simulink model "mavsim_manager_video"  (R2025a)
settings: Solver=ode45  StartTime=0.0  StopTime=inf  RelTol=1e-3  EnableMultiTasking=on
InitFcn:
  | param_chap11
undefined symbols (not defined in the file): autopilot, drawEnvironment, estimate_states, fym, gps, P, path_manager, path_planner_chap11, seguimiento, sensors, true_states
libraries: simulink x4
settings Model: Creator=beard  LastModifiedBy=anton
settings SolverCC: AlgebraicLoopSolver=TrustRegion
settings DataIOCC: LimitDataPoints=on  SaveFormat=Array  SignalLoggingSaveFormat=ModelDataLogs  ReturnWorkspaceOutputs=off
settings OptimizationCC: ExpressionDepthLimit=2147483647.0  InitFltsAndDblsToZero=on  LifeSpan=inf
settings DebuggingCC: UnderspecifiedInitializationDetection=Classic  MergeDetectMultiDrivingBlocksExec=none  SolverPrmCheckMsg=warning  FcnCallInpInsideContextMsg=warning  UnconnectedInputMsg=warning  UnconnectedOutputMsg=warning  UnconnectedLineMsg=warning  StateNameClashWarn=warning  SFUnexpectedBacktrackingDiag=warning  SFNoUnconditionalDefaultTransitionDiag=warning  ArithmeticOperatorsInVariantConditions=warning
settings HardwareCC: ProdBitPerPointer=32.0  ProdBitPerSizeT=32.0  ProdBitPerPtrDiffT=32.0  ProdLargestAtomicFloat=None  ProdIntDivRoundTo=Undefined  ProdEndianess=Unspecified  ProdWordSize=32.0  ProdHWDeviceType=32-bit Generic
settings ModelReferenceCC: EnableRefExpFcnMdlSchedulingChecks=on  PropagateSignalLabelsOutOfModel=off
settings SFSimCC: SimUseLocalCustomCode=off  SimParseCustomCode=off  CustomCodeUndefinedFunction=UseInterfaceOnly
settings RTWCC: RTWUseLocalCustomCode=off  GPUComputeCapability=3.5  DLArmComputeVersion=19.05
settings CodeAppCC: StateflowObjectComments=on
settings GRTTargetCC: TargetLangStandard=C89/C90 (ANSI)  CombineOutputUpdateFcns=off  GRTInterface=on
settings ConfigComp: CovMetricSettings=dw  CovSaveCumulativeToWorkspaceVar=on  CovSaveSingleToWorkspaceVar=on  CovExternalEMLEnable=off  CovSFcnEnable=off

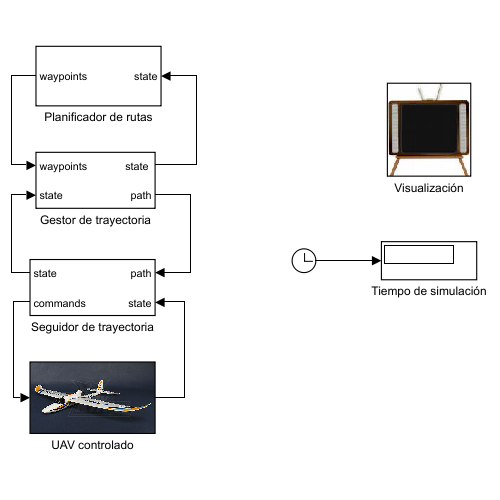
[thumbnail: Simulink's stored preview of the top-level diagram]
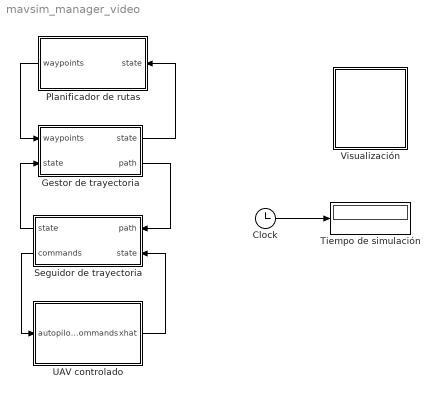
== system mavsim_manager_video ==
  Clock : Clock
  Gestor de trayectoria : Subsystem
  Planificador de rutas : Subsystem
  Seguidor de trayectoria : Subsystem
  Tiempo de simulación : Display
  UAV controlado : Subsystem
      mask Display: image(imread('uav.jpg'))
  Visualización : Subsystem
      mask Display: image(imread('tv.jpg'))
  wires:
  Clock/1 -> Tiempo de simulación/1
  Gestor de trayectoria/2(path) -> Seguidor de trayectoria/1(path)
  Seguidor de trayectoria/2(commands) -> UAV controlado/1(autopilot commands)
  UAV controlado/1(xhat) -> Seguidor de trayectoria/2(state)
  Seguidor de trayectoria/1("state ") -> Gestor de trayectoria/2(state)
  Planificador de rutas/1(waypoints) -> Gestor de trayectoria/1(waypoints)
  Gestor de trayectoria/1("state ") -> Planificador de rutas/1(state)

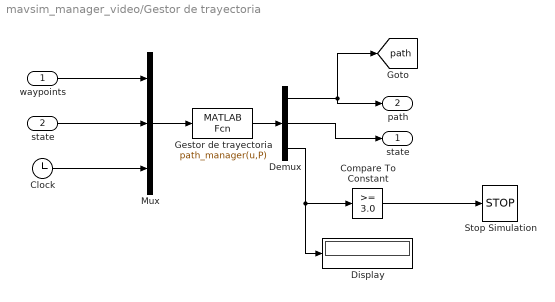
== system mavsim_manager_video/Gestor de trayectoria ==
  waypoints : Inport
  state : Inport  Port=2
  Clock : Clock
  Compare To Constant : simulink/Logic and Bit Operations/Compare To Constant  relop=>=  const=3.0  OutDataTypeStr=boolean
  Demux : Demux  Outputs=[13;17;1]
  Display : Display
  Gestor de trayectoria : MATLABFcn  MATLABFcn=path_manager(u,P)  OutputDimensions=31  SampleTime=P.Ts
  Mux : Mux  Inputs=3
  Stop Simulation : Stop
  "state " : Outport
  path : Outport  Port=2
  tag scope: path=global
  wires:
  Demux/2 -> "state "/1
  Demux/1 -> path/1, [path]
  Gestor de trayectoria/1 -> Demux/1
  waypoints/1 -> Mux/1
  state/1 -> Mux/2
  Clock/1 -> Mux/3
  Mux/1 -> Gestor de trayectoria/1
  Demux/3 -> Compare To Constant/1, Display/1
  Compare To Constant/1 -> Stop Simulation/1

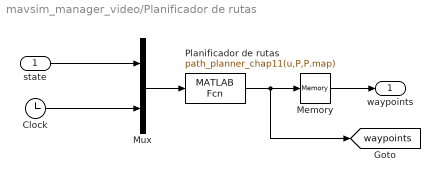
== system mavsim_manager_video/Planificador de rutas ==
  state : Inport
  Clock : Clock
  Memory : Memory
  Mux : Mux  Inputs=2
  Planificador de rutas : MATLABFcn  MATLABFcn=path_planner_chap11(u,P,P.map)  OutputDimensions=1+5*P.size_waypoint_array  SampleTime=100*P.Ts
  waypoints : Outport
  tag scope: waypoints=global
  wires:
  Mux/1 -> Planificador de rutas/1
  Clock/1 -> Mux/2
  state/1 -> Mux/1
  Planificador de rutas/1 -> Memory/1, [waypoints]
  Memory/1 -> waypoints/1

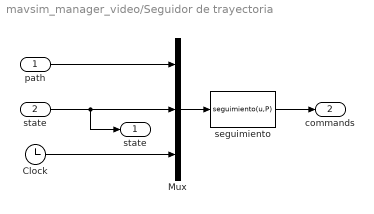
== system mavsim_manager_video/Seguidor de trayectoria ==
  path : Inport
  state : Inport  Port=2
  Clock : Clock
  Mux : Mux  Inputs=3
  seguimiento : MATLABFcn  MATLABFcn=seguimiento(u,P)  OutputDimensions=3  SampleTime=P.Ts
  "state " : Outport
  commands : Outport  Port=2
  wires:
  seguimiento/1 -> commands/1
  Mux/1 -> seguimiento/1
  path/1 -> Mux/1
  Clock/1 -> Mux/3
  state/1 -> Mux/2, "state "/1

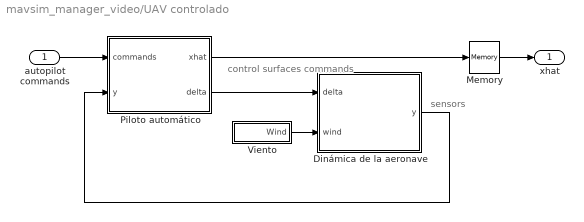
== system mavsim_manager_video/UAV controlado ==
  note: control surfaces
      | commands
  note: sensors
  autopilot commands : Inport
  Dinámica de la aeronave : Subsystem
      mask Display: image(imread('uav.jpg'))
  Memory : Memory
  Piloto automático : Subsystem
      mask Display: image(imread('pixfalcon.jpeg'))
  Viento : Subsystem
  xhat : Outport
  wires:
  Memory/1 -> xhat/1
  Piloto automático/1(xhat) -> Memory/1
  autopilot commands/1 -> Piloto automático/1(commands)
  Dinámica de la aeronave/1(y) -> Piloto automático/2(y)
  Piloto automático/2(delta) -> Dinámica de la aeronave/1(delta)
  Viento/1(Wind) -> Dinámica de la aeronave/2(wind)

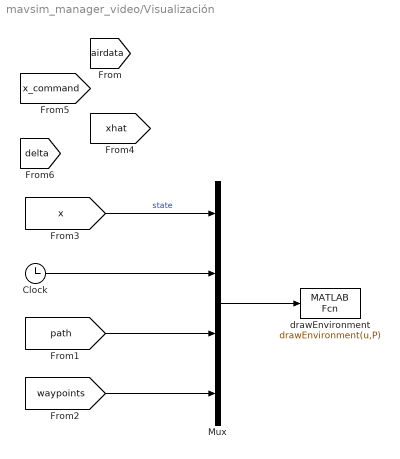
== system mavsim_manager_video/Visualización ==
  Clock : Clock
  Mux : Mux
  drawEnvironment : MATLABFcn  MATLABFcn=drawEnvironment(u,P)  OutputDimensions=0  SampleTime=0.1
  wires:
  Clock/1 -> Mux/2
  [x] -> Mux/1  "state"
  Mux/1 -> drawEnvironment/1
  [path] -> Mux/3
  [waypoints] -> Mux/4

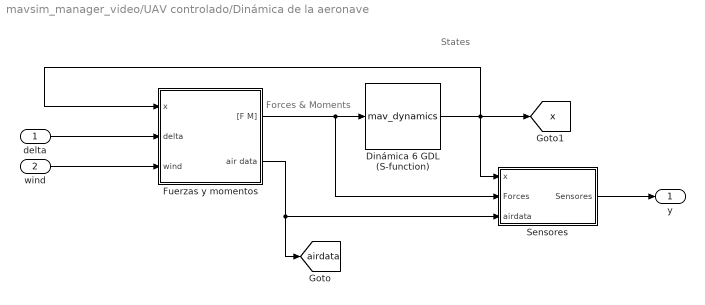
== system mavsim_manager_video/UAV controlado/Dinámica de la aeronave ==
  note: States
  note: Forces & Moments
  delta : Inport
  wind : Inport  Port=2
  Dinámica 6 GDL (S-function) : M-S-Function  FunctionName=mav_dynamics  Parameters=mass,Jx,Jy,Jz,Jxz,pn0,pe0,pd0,u0,v0,w0,phi0,theta0,psi0,p0,q0,r0  mask{mass=P.mass, Jx=P.Jx, Jy=P.Jy, Jz=P.Jz, Jxz=P.Jxz, pn0=P.pn0, pe0=P.pe0, pd0=P.pd0, u0=P.u0, v0=P.v0, w0=P.w0, phi0=P.phi0, theta0=P.theta0, psi0=P.psi0, p0=P.p0, q0=P.q0, r0=P.r0}
  Fuerzas y momentos : Subsystem
  Sensores : Subsystem
  y : Outport
  tag scope: airdata=global, x=global
  wires:
  wind/1 -> Fuerzas y momentos/3(wind)
  delta/1 -> Fuerzas y momentos/2(delta)
  Fuerzas y momentos/2(air data) -> Sensores/3(airdata), [airdata]
  Fuerzas y momentos/1("[F M]") -> Dinámica 6 GDL (S-function)/1, Sensores/2(Forces)
  Dinámica 6 GDL (S-function)/1 -> [x], Sensores/1(x), Fuerzas y momentos/1(x)
  Sensores/1(Sensores) -> y/1

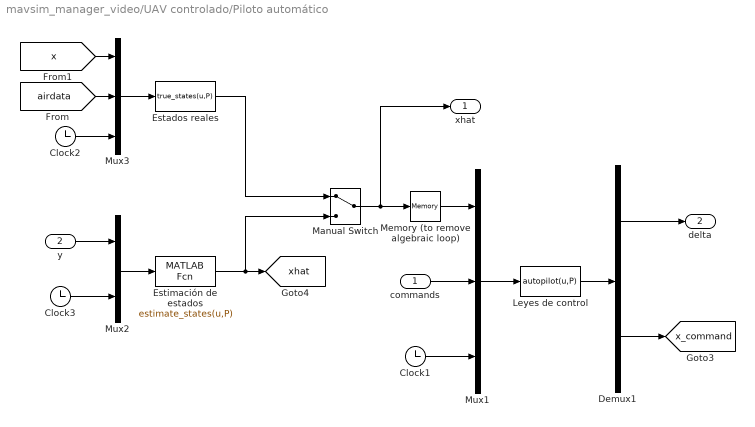
== system mavsim_manager_video/UAV controlado/Piloto automático ==
  commands : Inport
  y : Inport  Port=2
  Clock1 : Clock
  Clock2 : Clock
  Clock3 : Clock
  Demux1 : Demux  Outputs=[4;12]
  Estados reales : MATLABFcn  MATLABFcn=true_states(u,P)  OutputDimensions=19  SampleTime=P.Ts
  Estimación de estados : MATLABFcn  MATLABFcn=estimate_states(u,P)  OutputDimensions=19  SampleTime=P.Ts
  Leyes de control : MATLABFcn  MATLABFcn=autopilot(u,P)  OutputDimensions=4+12  SampleTime=P.Ts
  Manual Switch : ManualSwitch
  Memory (to remove algebraic loop) : Memory
  Mux1 : Mux  Inputs=3
  Mux2 : Mux  Inputs=2
  Mux3 : Mux  Inputs=3
  xhat : Outport
  delta : Outport  Port=2
  tag scope: x_command=global, xhat=global
  wires:
  Estimación de estados/1 -> [xhat], Manual Switch/2
  Clock3/1 -> Mux2/2
  Clock2/1 -> Mux3/3
  Clock1/1 -> Mux1/3
  [x] -> Mux3/1
  [airdata] -> Mux3/2
  Mux3/1 -> Estados reales/1
  Estados reales/1 -> Manual Switch/1
  Manual Switch/1 -> xhat/1, Memory (to remove algebraic loop)/1
  Memory (to remove algebraic loop)/1 -> Mux1/1
  y/1 -> Mux2/1
  Mux2/1 -> Estimación de estados/1
  commands/1 -> Mux1/2
  Demux1/2 -> [x_command]
  Demux1/1 -> delta/1
  Leyes de control/1 -> Demux1/1
  Mux1/1 -> Leyes de control/1

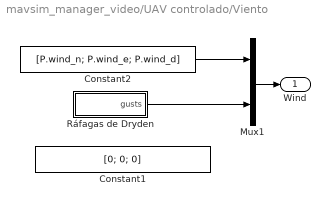
== system mavsim_manager_video/UAV controlado/Viento ==
  Constant1 : Constant  Value=[0; 0; 0]
  Constant2 : Constant  Value=[P.wind_n; P.wind_e; P.wind_d]
  Mux1 : Mux  Inputs=2
  Ráfagas de Dryden : Subsystem
  Wind : Outport
  wires:
  Mux1/1 -> Wind/1
  Constant2/1 -> Mux1/1
  Ráfagas de Dryden/1(gusts) -> Mux1/2

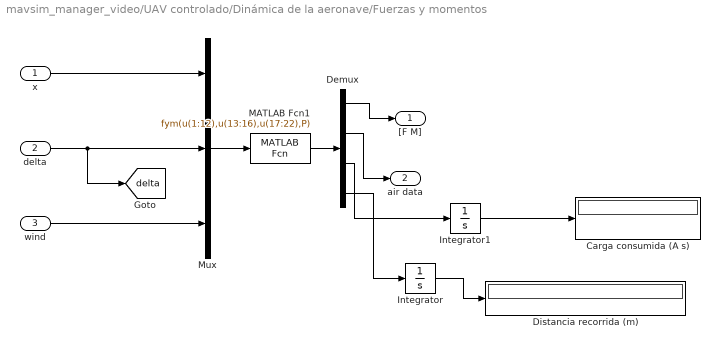
== system mavsim_manager_video/UAV controlado/Dinámica de la aeronave/Fuerzas y momentos ==
  x : Inport
  delta : Inport  Port=2
  wind : Inport  Port=3
  Carga consumida (A s) : Display
  Demux : Demux  Outputs=[6;6;1;1]
  Distancia recorrida (m) : Display
      settings: Decimation=4
  Integrator : Integrator
  Integrator1 : Integrator
  MATLAB Fcn1 : MATLABFcn  MATLABFcn=fym(u(1:12),u(13:16),u(17:22),P)  OutputDimensions=14
  Mux : Mux  Inputs=3
  "[F M]" : Outport
  air data : Outport  Port=2
  tag scope: delta=global
  wires:
  Demux/2 -> air data/1
  Mux/1 -> MATLAB Fcn1/1
  Demux/1 -> "[F M]"/1
  MATLAB Fcn1/1 -> Demux/1
  wind/1 -> Mux/3
  delta/1 -> Mux/2, [delta]
  x/1 -> Mux/1
  Demux/3 -> Integrator1/1
  Demux/4 -> Integrator/1
  Integrator/1 -> Distancia recorrida (m)/1
  Integrator1/1 -> Carga consumida (A s)/1

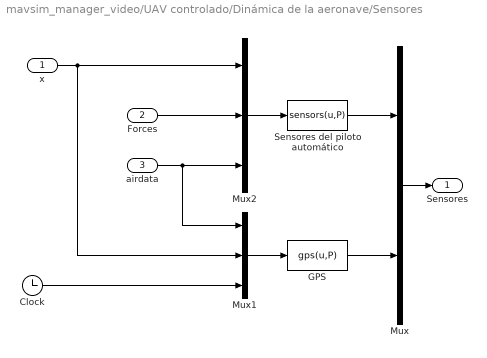
== system mavsim_manager_video/UAV controlado/Dinámica de la aeronave/Sensores ==
  x : Inport
  Forces : Inport  Port=2
  airdata : Inport  Port=3
  Clock : Clock
  GPS : MATLABFcn  MATLABFcn=gps(u,P)  OutputDimensions=5  SampleTime=P.Ts_gps
  Mux : Mux  Inputs=2
  Mux1 : Mux  Inputs=3
  Mux2 : Mux  Inputs=3
  Sensores del piloto automático : MATLABFcn  MATLABFcn=sensors(u,P)  OutputDimensions=8  SampleTime=P.Ts
  Sensores : Outport
  wires:
  x/1 -> Mux1/2, Mux2/1
  Mux/1 -> Sensores/1
  airdata/1 -> Mux1/1, Mux2/3
  Forces/1 -> Mux2/2
  Mux2/1 -> Sensores del piloto automático/1
  Clock/1 -> Mux1/3
  Mux1/1 -> GPS/1
  GPS/1 -> Mux/2
  Sensores del piloto automático/1 -> Mux/1

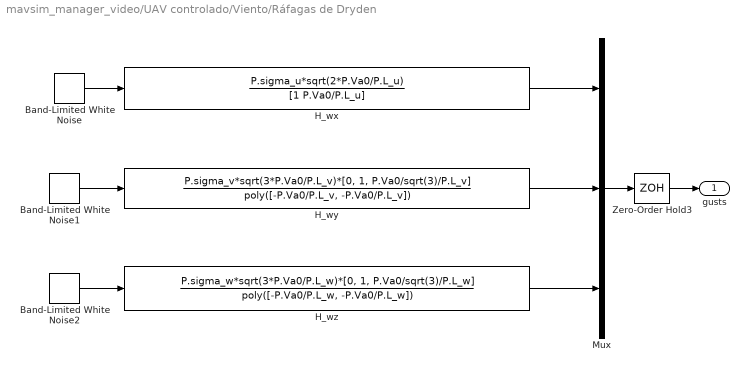
== system mavsim_manager_video/UAV controlado/Viento/Ráfagas de Dryden ==
  Band-Limited White Noise : simulink/Sources/Band-Limited White Noise  Cov=[1]  Ts=P.Ts  seed=[23341]
  Band-Limited White Noise1 : simulink/Sources/Band-Limited White Noise  Cov=[1]  Ts=P.Ts  seed=[23341]
  Band-Limited White Noise2 : simulink/Sources/Band-Limited White Noise  Cov=[1]  Ts=P.Ts  seed=[23341]
  H_wx : TransferFcn  Numerator=P.sigma_u*sqrt(2*P.Va0/P.L_u)  Denominator=[1 P.Va0/P.L_u]
  H_wy : TransferFcn  Numerator=P.sigma_v*sqrt(3*P.Va0/P.L_v)*[0, 1, P.Va0/sqrt(3)/P.L_v]  Denominator=poly([-P.Va0/P.L_v, -P.Va0/P.L_v])
  H_wz : TransferFcn  Numerator=P.sigma_w*sqrt(3*P.Va0/P.L_w)*[0, 1, P.Va0/sqrt(3)/P.L_w]  Denominator=poly([-P.Va0/P.L_w, -P.Va0/P.L_w])
  Mux : Mux  Inputs=3
  Zero-Order Hold3 : ZeroOrderHold  SampleTime=P.Ts
  gusts : Outport
  wires:
  H_wx/1 -> Mux/1
  Band-Limited White Noise/1 -> H_wx/1
  H_wy/1 -> Mux/2
  Band-Limited White Noise1/1 -> H_wy/1
  H_wz/1 -> Mux/3
  Band-Limited White Noise2/1 -> H_wz/1
  Mux/1 -> Zero-Order Hold3/1
  Zero-Order Hold3/1 -> gusts/1
